simulink model "hdlcoder_bitops_eml"  (R2026a)
settings: Solver=FixedStepDiscrete  StopTime=10  FixedStep=1
settings Model: Creator=The MathWorks, Inc.  LastModifiedBy=The MathWorks, Inc.
settings DataIOCC: SaveFormat=StructureWithTime
settings OptimizationCC: ConditionallyExecuteInputs=off  InitFltsAndDblsToZero=on
settings DebuggingCC: AlgebraicLoopMsg=error  UnderspecifiedInitializationDetection=Classic  MultiTaskDSMMsg=warning  MultiTaskCondExecSysMsg=none  SingleTaskRateTransMsg=error
settings HardwareCC: ProdHWDeviceType=ASIC/FPGA
settings GRTTargetCC: CombineOutputUpdateFcns=off  GRTInterface=on

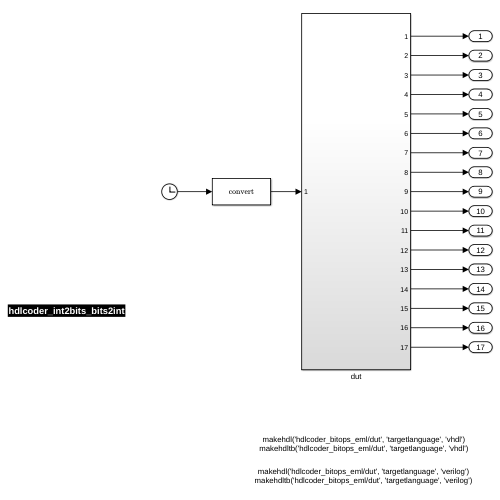
[thumbnail: Simulink's stored preview of the top-level diagram]
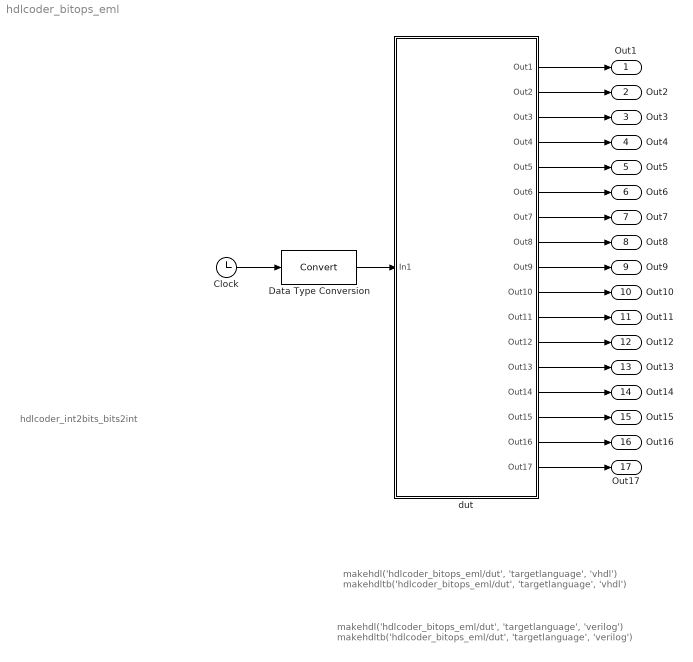
== system hdlcoder_bitops_eml ==
  note: makehdl('hdlcoder_bitops_eml/dut', 'targetlanguage', 'vhdl')
      | makehdltb('hdlcoder_bitops_eml/dut', 'targetlanguage', 'vhdl')
  note: makehdl('hdlcoder_bitops_eml/dut', 'targetlanguage', 'verilog')
      | makehdltb('hdlcoder_bitops_eml/dut', 'targetlanguage', 'verilog')
  note: hdlcoder_int2bits_bits2int
  Clock : Clock
  Data Type Conversion : DataTypeConversion  SaturateOnIntegerOverflow=off  RndMeth=Floor
  dut : Subsystem
  Out1 : Outport
  Out2 : Outport  Port=2
  Out3 : Outport  Port=3
  Out4 : Outport  Port=4
  Out5 : Outport  Port=5
  Out6 : Outport  Port=6
  Out7 : Outport  Port=7
  Out8 : Outport  Port=8
  Out9 : Outport  Port=9
  Out10 : Outport  Port=10
  Out11 : Outport  Port=11
  Out12 : Outport  Port=12
  Out13 : Outport  Port=13
  Out14 : Outport  Port=14
  Out15 : Outport  Port=15
  Out16 : Outport  Port=16
  Out17 : Outport  Port=17
  wires:
  Clock/1 -> Data Type Conversion/1
  Data Type Conversion/1 -> dut/1(In1)
  dut/1(Out1) -> Out1/1
  dut/2(Out2) -> Out2/1
  dut/3(Out3) -> Out3/1
  dut/4(Out4) -> Out4/1
  dut/5(Out5) -> Out5/1
  dut/6(Out6) -> Out6/1
  dut/7(Out7) -> Out7/1
  dut/8(Out8) -> Out8/1
  dut/9(Out9) -> Out9/1
  dut/10(Out10) -> Out10/1
  dut/11(Out11) -> Out11/1
  dut/12(Out12) -> Out12/1
  dut/13(Out13) -> Out13/1
  dut/14(Out14) -> Out14/1
  dut/15(Out15) -> Out15/1
  dut/16(Out16) -> Out16/1
  dut/17(Out17) -> Out17/1

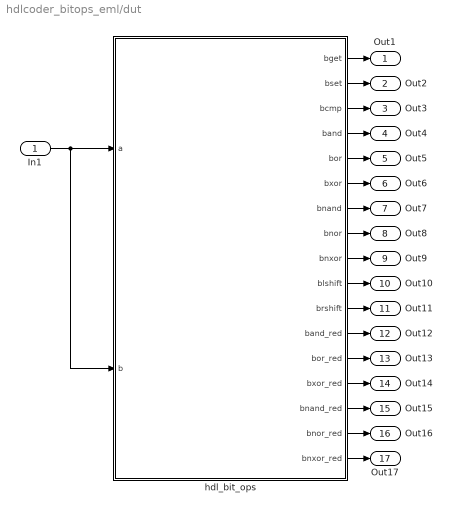
== system hdlcoder_bitops_eml/dut ==
  In1 : Inport
  hdl_bit_ops : MATLAB Function  TreatAsAtomicUnit=on
  Out1 : Outport
  Out2 : Outport  Port=2
  Out3 : Outport  Port=3
  Out4 : Outport  Port=4
  Out5 : Outport  Port=5
  Out6 : Outport  Port=6
  Out7 : Outport  Port=7
  Out8 : Outport  Port=8
  Out9 : Outport  Port=9
  Out10 : Outport  Port=10
  Out11 : Outport  Port=11
  Out12 : Outport  Port=12
  Out13 : Outport  Port=13
  Out14 : Outport  Port=14
  Out15 : Outport  Port=15
  Out16 : Outport  Port=16
  Out17 : Outport  Port=17
  wires:
  In1/1 -> hdl_bit_ops/2(b), hdl_bit_ops/1(a)
  hdl_bit_ops/1(bget) -> Out1/1
  hdl_bit_ops/2(bset) -> Out2/1
  hdl_bit_ops/3(bcmp) -> Out3/1
  hdl_bit_ops/4(band) -> Out4/1
  hdl_bit_ops/5(bor) -> Out5/1
  hdl_bit_ops/6(bxor) -> Out6/1
  hdl_bit_ops/7(bnand) -> Out7/1
  hdl_bit_ops/8(bnor) -> Out8/1
  hdl_bit_ops/9(bnxor) -> Out9/1
  hdl_bit_ops/10(blshift) -> Out10/1
  hdl_bit_ops/11(brshift) -> Out11/1
  hdl_bit_ops/12(band_red) -> Out12/1
  hdl_bit_ops/13(bor_red) -> Out13/1
  hdl_bit_ops/14(bxor_red) -> Out14/1
  hdl_bit_ops/15(bnand_red) -> Out15/1
  hdl_bit_ops/16(bnor_red) -> Out16/1
  hdl_bit_ops/17(bnxor_red) -> Out17/1

== matlab function hdlcoder_bitops_eml/dut/hdl_bit_ops ==
  settings: fimath=|
      | fimath(...
      | 'RoundMode', 'floor',...
      | 'OverflowMode', 'saturate',...
      | 'ProductMode', 'FullPrecision', 'ProductWordLength', 32,...
      | 'SumMode', 'FullPrecision', 'SumWordLength', 32,...
      | 'CastBeforeSum', true)
  data: a input fixdt(0,31,0); b input fixdt(0,31,0); bget output; bset output; bcmp output; band output; bor output; bxor output; bnand output; bnor output; bnxor output; blshift output; brshift output; band_red output; bor_red output; bxor_red output; bnand_red output; bnor_red output; bnxor_red output
function [...
    bget, bset, bcmp,...
    band, bor, bxor, ...
    bnand, bnor, bnxor, ...
    blshift, brshift,  ...
    band_red, bor_red, bxor_red, ...
    bnand_red, bnor_red, bnxor_red] = fcn(a,b)


% BITGET
% get bit at position of fixed point input var 'a'
% this uses slice operator in HDL
bget = bitsliceget(a,2,2);

% BITCLEAR
% clear bit at position 3 and compute new value into 't2'
t2 = bitset(a,3,0);

% BITSET
% now set bit4 in t2
% you need to assign the result back to 't2' to update the variable
bset = bitset(t2,4,1);

% BITCMP
bcmp = bitcmp(a);

% BITAND
band = bitand(a,b);
% BITOR
bor = bitor(a,b);
% BITXOR
bxor = bitxor(a,b);

% BITNAND
bnand = bitcmp(bitand(a,b));
% BITNOR
bnor = bitcmp(bitor(a,b));
% NOT BITXOR
bnxor = bitcmp(bitxor(a,b));

% BITSHIFT
% multitply by 2
blshift = bitsll(a,1); 
% divide by 2
brshift = bitsrl(a,1); 

% AND, XOR, OR REDUCTION 
band_red = bitandreduce(a, 10, 5);
bxor_red = bitxorreduce(a, 10, 5);
bor_red = bitorreduce(a, 10, 5);

% NAND, NOR, NOT XOR, REDUCTION 
bnand_red = bitcmp(band_red);
bnxor_red = bitcmp(bxor_red);
bnor_red = bitcmp(bor_red);
